simulink model "ex5_12"  (R2026a)
settings: Solver=FixedStepAuto  StopTime=20  FixedStep=0.001
values from neighbouring files (symbols this model uses):
  c = C(i)    [ex5_12.m]
  k = K(j)    [ex5_12.m]
settings Model: Creator=User  LastModifiedBy=User

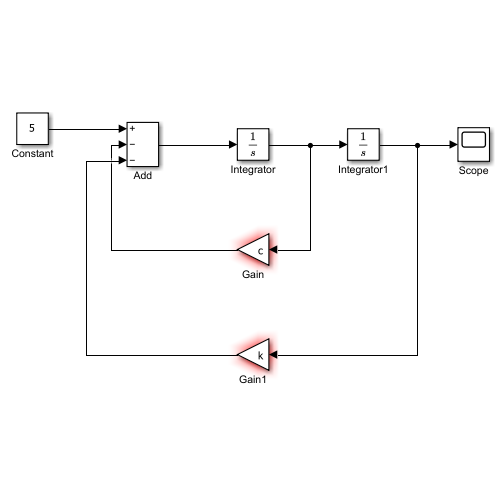
[thumbnail: Simulink's stored preview of the top-level diagram]
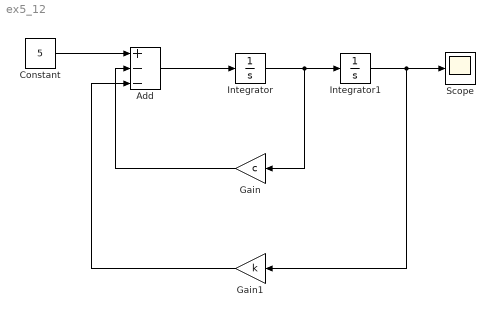
== system ex5_12 ==
  Add : Sum  Inputs=+--
  Constant : Constant  Value=5
  Gain : Gain  Gain=c
  Gain1 : Gain  Gain=k
  Integrator : Integrator
  Integrator1 : Integrator
  Scope : Scope
  wires:
  Constant/1 -> Add/1
  Add/1 -> Integrator/1
  Integrator/1 -> Gain/1, Integrator1/1
  Integrator1/1 -> Gain1/1, Scope/1
  Gain/1 -> Add/2
  Gain1/1 -> Add/3
